simulink model "Point1"  (R2025b)
settings: Solver=VariableStepAuto  StartTime=0.0  StopTime=10.0  RelTol=1e-3
settings Model: Creator=user  LastModifiedBy=user

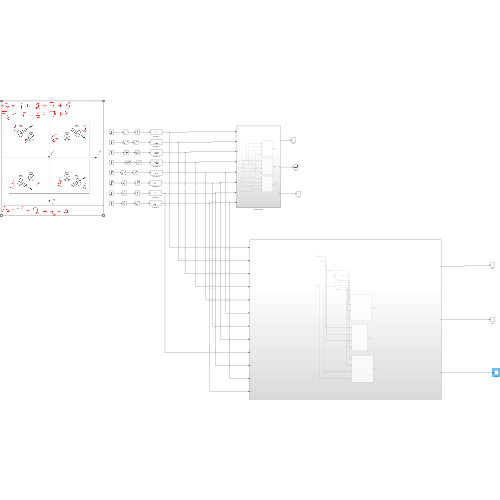
[thumbnail: Simulink's stored preview of the top-level diagram]
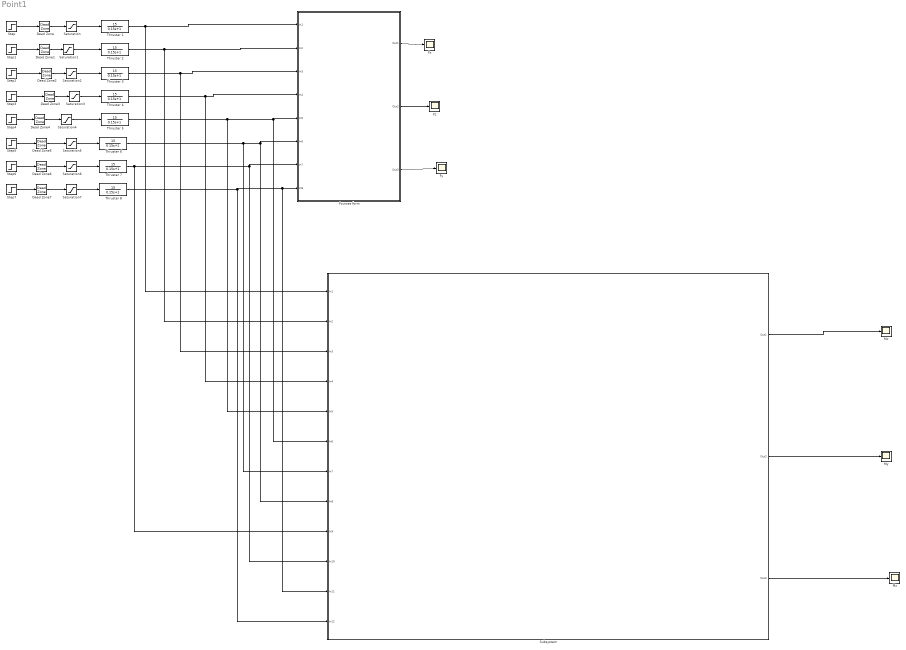
== system Point1 ==
  Dead Zone{,1..7} (8 alike) : DeadZone
  Fources form : Subsystem
  Fx : Scope
      settings: ActiveDisplayYMinimum=-2.6516504294495529  ActiveDisplayYMaximum=23.86485386504598
  Fy : Scope
      settings: ActiveDisplayYMinimum=-3.7499999999999991  ActiveDisplayYMaximum=33.75
  Fz : Scope
      settings: ActiveDisplayYMinimum=-1  ActiveDisplayYMaximum=1  DataLoggingVariableName=ScopeData2
  Mx : Scope
      settings: ActiveDisplayYMinimum=-1  ActiveDisplayYMaximum=1  DataLoggingVariableName=ScopeData3
  My : Scope
      settings: ActiveDisplayYMinimum=-1  ActiveDisplayYMaximum=1  DataLoggingVariableName=ScopeData4
  Mz : Scope
      settings: ActiveDisplayYMinimum=-1  ActiveDisplayYMaximum=1  DataLoggingVariableName=ScopeData5
  Saturation{,1..7} (8 alike) : Saturate  UpperLimit=10  LowerLimit=-10
  Step{,1..7} (8 alike) : Step  SampleTime=0
  Subsystem : Subsystem
  Thruster {1..8} (8 alike) : TransferFcn  Numerator=[15]  Denominator=[0.15 1]
  wires:
  Dead Zone/1 -> Saturation/1
  Step/1 -> Dead Zone/1
  Step1/1 -> Dead Zone1/1
  Dead Zone1/1 -> Saturation1/1
  Step2/1 -> Dead Zone2/1
  Dead Zone2/1 -> Saturation2/1
  Step3/1 -> Dead Zone3/1
  Dead Zone3/1 -> Saturation3/1
  Step4/1 -> Dead Zone4/1
  Dead Zone4/1 -> Saturation4/1
  Step5/1 -> Dead Zone5/1
  Dead Zone5/1 -> Saturation5/1
  Step6/1 -> Dead Zone6/1
  Dead Zone6/1 -> Saturation6/1
  Step7/1 -> Dead Zone7/1
  Dead Zone7/1 -> Saturation7/1
  Saturation/1 -> Thruster 1/1
  Saturation1/1 -> Thruster 2/1
  Saturation2/1 -> Thruster 3/1
  Saturation3/1 -> Thruster 4/1
  Saturation4/1 -> Thruster 5/1
  Saturation7/1 -> Thruster 8/1
  Saturation6/1 -> Thruster 7/1
  Saturation5/1 -> Thruster 6/1
  Thruster 1/1 -> Subsystem/1(In1), Fources form/1(In1)
  Thruster 2/1 -> Subsystem/2(In2), Fources form/2(In2)
  Thruster 3/1 -> Subsystem/3(In3), Fources form/3(In3)
  Thruster 5/1 -> Subsystem/5(In5), Subsystem/6(In6), Fources form/5(In5)
  Thruster 6/1 -> Subsystem/7(In7), Subsystem/8(In8), Fources form/6(In6)
  Thruster 7/1 -> Subsystem/9(In9), Subsystem/10(In10), Fources form/7(In7)
  Thruster 8/1 -> Subsystem/12(In12), Subsystem/11(In11), Fources form/8(In8)
  Fources form/1(Out1) -> Fx/1
  Thruster 4/1 -> Subsystem/4(In4), Fources form/4(In4)
  Subsystem/1(Out1) -> Mx/1
  Subsystem/3(Out3) -> Mz/1
  Subsystem/2(Out2) -> My/1
  Fources form/2(Out2) -> Fz/1
  Fources form/3(Out3) -> Fy/1

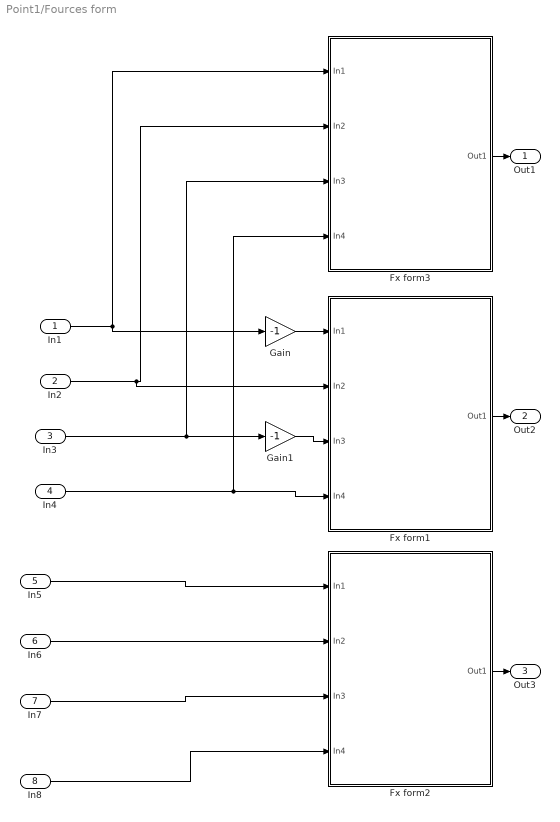
== system Point1/Fources form ==
  In1 : Inport
  In2 : Inport  Port=2
  In3 : Inport  Port=3
  In4 : Inport  Port=4
  In5 : Inport  Port=5
  In6 : Inport  Port=6
  In7 : Inport  Port=7
  In8 : Inport  Port=8
  Fx form1 : Subsystem
  Fx form2 : Subsystem
  Fx form3 : Subsystem
  Gain : Gain  Gain=-1
  Gain1 : Gain  Gain=-1
  Out1 : Outport
  Out2 : Outport  Port=2
  Out3 : Outport  Port=3
  wires:
  In4/1 -> Fx form1/4(In4), Fx form3/4(In4)
  In3/1 -> Gain1/1, Fx form3/3(In3)
  In1/1 -> Fx form3/1(In1), Gain/1
  Fx form2/1(Out1) -> Out3/1
  Fx form3/1(Out1) -> Out1/1
  Fx form1/1(Out1) -> Out2/1
  In2/1 -> Fx form1/2(In2), Fx form3/2(In2)
  In5/1 -> Fx form2/1(In1)
  In6/1 -> Fx form2/2(In2)
  In7/1 -> Fx form2/3(In3)
  In8/1 -> Fx form2/4(In4)
  Gain/1 -> Fx form1/1(In1)
  Gain1/1 -> Fx form1/3(In3)

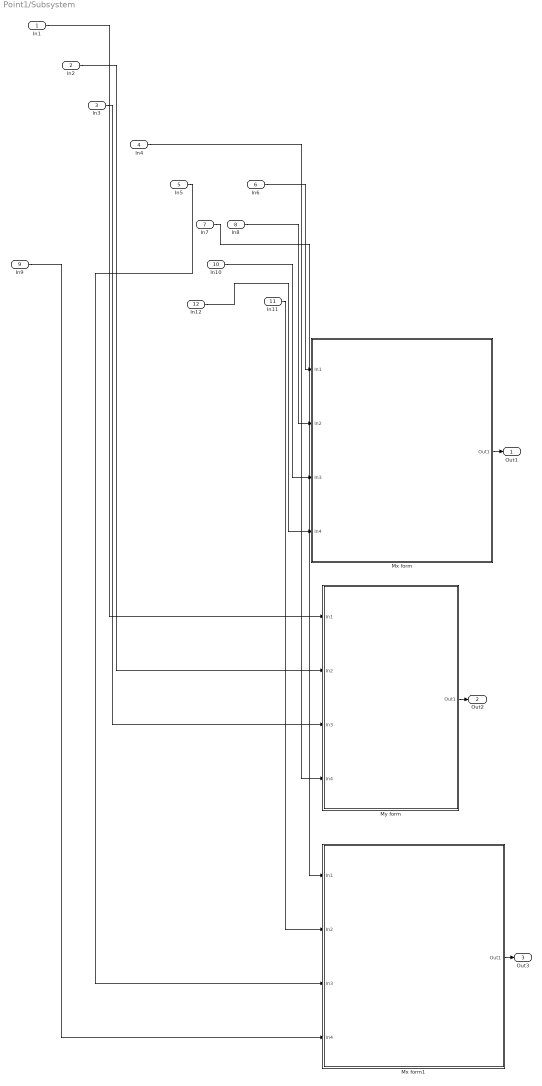
== system Point1/Subsystem ==
  In1 : Inport
  In2 : Inport  Port=2
  In3 : Inport  Port=3
  In4 : Inport  Port=4
  In5 : Inport  Port=5
  In6 : Inport  Port=6
  In7 : Inport  Port=7
  In8 : Inport  Port=8
  In9 : Inport  Port=9
  In10 : Inport  Port=10
  In11 : Inport  Port=11
  In12 : Inport  Port=12
  Mx form : Subsystem
  Mx form1 : Subsystem
  My form : Subsystem
  Out1 : Outport
  Out2 : Outport  Port=2
  Out3 : Outport  Port=3
  wires:
  In11/1 -> Mx form1/2(In2)
  In3/1 -> My form/3(In3)
  In6/1 -> Mx form/1(In1)
  In1/1 -> My form/1(In1)
  In5/1 -> Mx form1/3(In3)
  In12/1 -> Mx form/4(In4)
  In8/1 -> Mx form/2(In2)
  In10/1 -> Mx form/3(In3)
  In2/1 -> My form/2(In2)
  In4/1 -> My form/4(In4)
  In7/1 -> Mx form1/1(In1)
  In9/1 -> Mx form1/4(In4)
  Mx form/1(Out1) -> Out1/1
  Mx form1/1(Out1) -> Out3/1
  My form/1(Out1) -> Out2/1

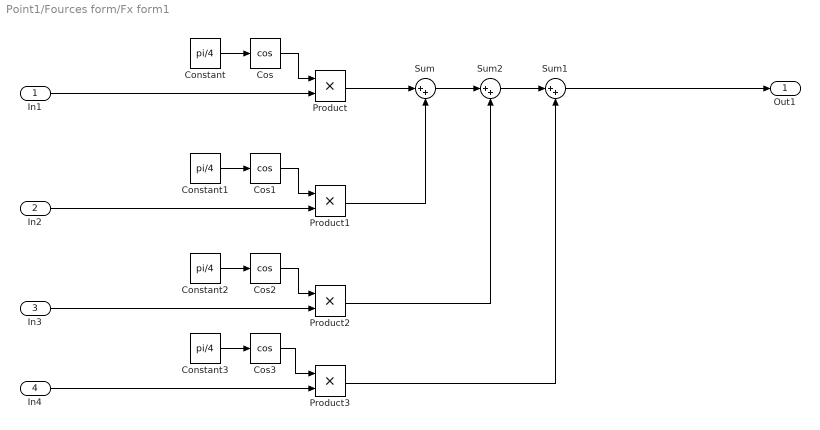
== system Point1/Fources form/Fx form1 ==
  In1 : Inport
  In2 : Inport  Port=2
  In3 : Inport  Port=3
  In4 : Inport  Port=4
  Constant{,1..3} (4 alike) : Constant  Value=pi/4
  Cos{,1..3} (4 alike) : Trigonometry  Operator=cos
  Product{,1..3} (4 alike) : Product
  Sum : Sum  Inputs=|++
  Sum1 : Sum  Inputs=|++
  Sum2 : Sum  Inputs=|++
  Out1 : Outport
  wires:
  Product/1 -> Sum/1
  Cos3/1 -> Product3/1
  Cos2/1 -> Product2/1
  Constant3/1 -> Cos3/1
  Constant2/1 -> Cos2/1
  Constant1/1 -> Cos1/1
  Cos1/1 -> Product1/1
  Constant/1 -> Cos/1
  In4/1 -> Product3/2
  Product1/1 -> Sum/2
  Cos/1 -> Product/1
  In3/1 -> Product2/2
  Sum1/1 -> Out1/1
  In1/1 -> Product/2
  In2/1 -> Product1/2
  Sum/1 -> Sum2/1
  Sum2/1 -> Sum1/1
  Product2/1 -> Sum2/2
  Product3/1 -> Sum1/2

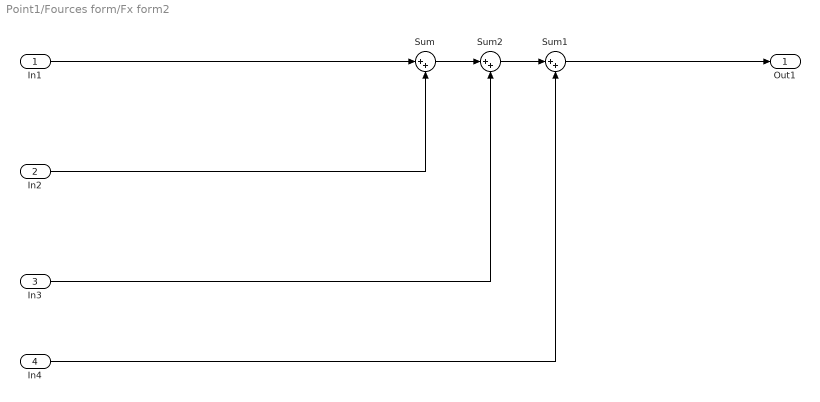
== system Point1/Fources form/Fx form2 ==
  In1 : Inport
  In2 : Inport  Port=2
  In3 : Inport  Port=3
  In4 : Inport  Port=4
  Sum : Sum  Inputs=|++
  Sum1 : Sum  Inputs=|++
  Sum2 : Sum  Inputs=|++
  Out1 : Outport
  wires:
  In1/1 -> Sum/1
  Sum1/1 -> Out1/1
  Sum/1 -> Sum2/1
  Sum2/1 -> Sum1/1
  In3/1 -> Sum2/2
  In4/1 -> Sum1/2
  In2/1 -> Sum/2

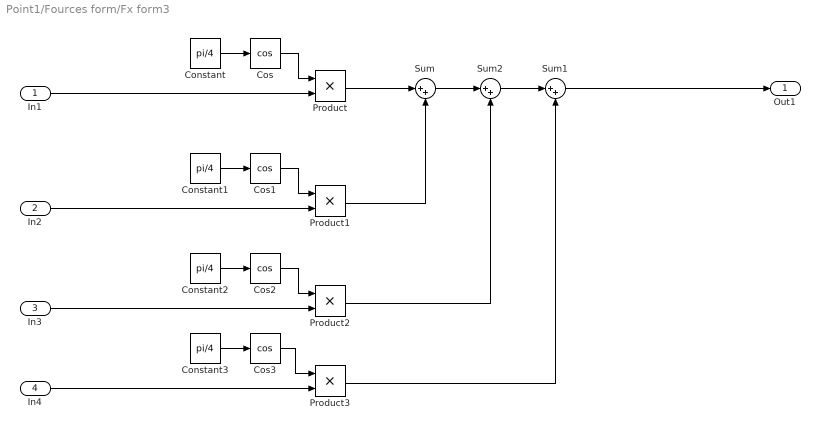
== system Point1/Fources form/Fx form3 ==
  In1 : Inport
  In2 : Inport  Port=2
  In3 : Inport  Port=3
  In4 : Inport  Port=4
  Constant{,1..3} (4 alike) : Constant  Value=pi/4
  Cos{,1..3} (4 alike) : Trigonometry  Operator=cos
  Product{,1..3} (4 alike) : Product
  Sum : Sum  Inputs=|++
  Sum1 : Sum  Inputs=|++
  Sum2 : Sum  Inputs=|++
  Out1 : Outport
  wires:
  Product/1 -> Sum/1
  Cos3/1 -> Product3/1
  Cos2/1 -> Product2/1
  Constant3/1 -> Cos3/1
  Constant2/1 -> Cos2/1
  Constant1/1 -> Cos1/1
  Cos1/1 -> Product1/1
  Constant/1 -> Cos/1
  In4/1 -> Product3/2
  Product1/1 -> Sum/2
  Cos/1 -> Product/1
  In3/1 -> Product2/2
  Sum1/1 -> Out1/1
  In1/1 -> Product/2
  In2/1 -> Product1/2
  Sum/1 -> Sum2/1
  Sum2/1 -> Sum1/1
  Product2/1 -> Sum2/2
  Product3/1 -> Sum1/2

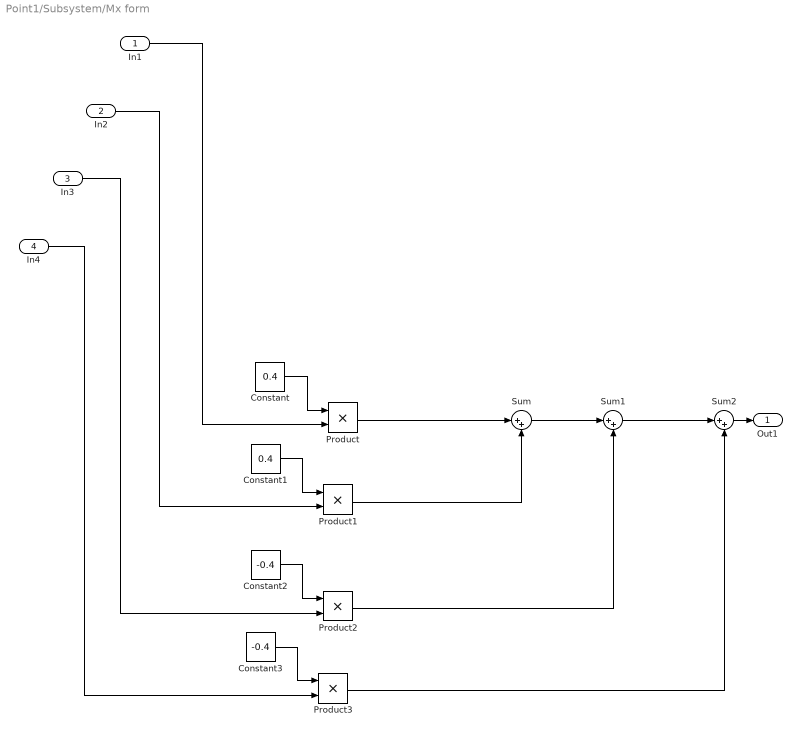
== system Point1/Subsystem/Mx form ==
  In1 : Inport
  In2 : Inport  Port=2
  In3 : Inport  Port=3
  In4 : Inport  Port=4
  Constant : Constant  Value=0.4
  Constant1 : Constant  Value=0.4
  Constant2 : Constant  Value=-0.4
  Constant3 : Constant  Value=-0.4
  Product{,1..3} (4 alike) : Product
  Sum : Sum  Inputs=|++
  Sum1 : Sum  Inputs=|++
  Sum2 : Sum  Inputs=|++
  Out1 : Outport
  wires:
  In2/1 -> Product1/2
  Product2/1 -> Sum1/2
  Constant/1 -> Product/1
  Constant1/1 -> Product1/1
  Constant3/1 -> Product3/1
  Sum1/1 -> Sum2/1
  Constant2/1 -> Product2/1
  Product/1 -> Sum/1
  Product3/1 -> Sum2/2
  In1/1 -> Product/2
  Sum/1 -> Sum1/1
  Product1/1 -> Sum/2
  In4/1 -> Product3/2
  Sum2/1 -> Out1/1
  In3/1 -> Product2/2

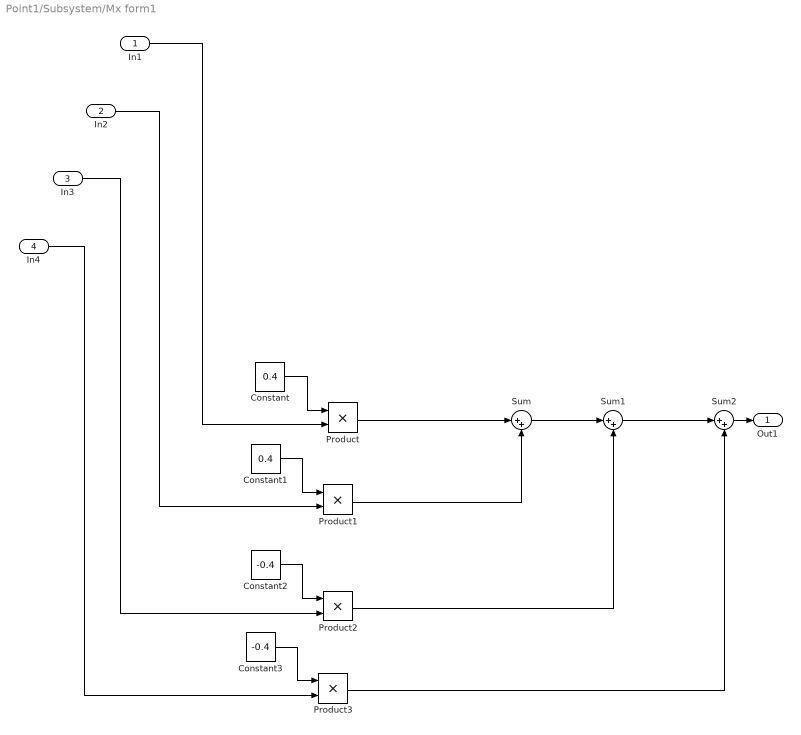
== system Point1/Subsystem/Mx form1 ==
  In1 : Inport
  In2 : Inport  Port=2
  In3 : Inport  Port=3
  In4 : Inport  Port=4
  Constant : Constant  Value=0.4
  Constant1 : Constant  Value=0.4
  Constant2 : Constant  Value=-0.4
  Constant3 : Constant  Value=-0.4
  Product{,1..3} (4 alike) : Product
  Sum : Sum  Inputs=|++
  Sum1 : Sum  Inputs=|++
  Sum2 : Sum  Inputs=|++
  Out1 : Outport
  wires:
  In2/1 -> Product1/2
  Product2/1 -> Sum1/2
  Constant/1 -> Product/1
  Constant1/1 -> Product1/1
  Constant3/1 -> Product3/1
  Sum1/1 -> Sum2/1
  Constant2/1 -> Product2/1
  Product/1 -> Sum/1
  Product3/1 -> Sum2/2
  In1/1 -> Product/2
  Sum/1 -> Sum1/1
  Product1/1 -> Sum/2
  In4/1 -> Product3/2
  Sum2/1 -> Out1/1
  In3/1 -> Product2/2

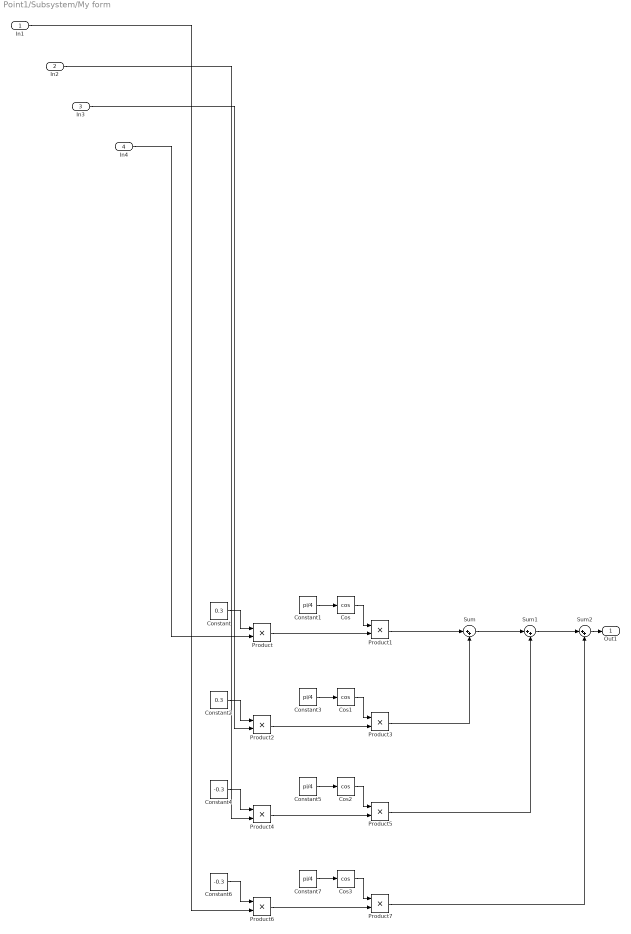
== system Point1/Subsystem/My form ==
  In1 : Inport
  In2 : Inport  Port=2
  In3 : Inport  Port=3
  In4 : Inport  Port=4
  Constant : Constant  Value=0.3
  Constant{1,3,5,7} (4 alike) : Constant  Value=pi/4
  Constant2 : Constant  Value=0.3
  Constant4 : Constant  Value=-0.3
  Constant6 : Constant  Value=-0.3
  Cos{,1..3} (4 alike) : Trigonometry  Operator=cos
  Product{,1..7} (8 alike) : Product
  Sum : Sum  Inputs=|++
  Sum1 : Sum  Inputs=|++
  Sum2 : Sum  Inputs=|++
  Out1 : Outport
  wires:
  Constant6/1 -> Product6/1
  Product2/1 -> Product3/2
  Product5/1 -> Sum1/2
  Constant/1 -> Product/1
  Product/1 -> Product1/2
  Constant7/1 -> Cos3/1
  Sum1/1 -> Sum2/1
  Product3/1 -> Sum/2
  Product7/1 -> Sum2/2
  Cos1/1 -> Product3/1
  Cos2/1 -> Product5/1
  Constant5/1 -> Cos2/1
  Cos3/1 -> Product7/1
  Product6/1 -> Product7/2
  Product1/1 -> Sum/1
  Cos/1 -> Product1/1
  Constant3/1 -> Cos1/1
  Product4/1 -> Product5/2
  In3/1 -> Product2/2
  Constant2/1 -> Product2/1
  Constant4/1 -> Product4/1
  Sum/1 -> Sum1/1
  Constant1/1 -> Cos/1
  In4/1 -> Product/2
  In2/1 -> Product4/2
  Sum2/1 -> Out1/1
  In1/1 -> Product6/2
